simulink model "nav_closed_loop"  (R2026a)
settings: Solver=FixedStepDiscrete  StartTime=0  StopTime=182.32  FixedStep=Ts
values from neighbouring files (symbols this model uses):
  P = nav_params(cfg, root)    [build_nav_simulink.m]    (also in nav_ablation.m; nav_figures.m = PP; nav_main.m; nav_study.m)
  trk = struct('N', TR.trk.N, 'ds', TR.trk.ds, 'L', TR.trk.L, 'x', TR.trk.x, 'y', TR.trk.y,               'psi', TR.trk.psi, 'kap', TR.trk.kap)    [build_nav_simulink.m]    (also in nav_ablation.m = TR.trk; nav_figures.m = TR.trk; end; nav_main.m = TR.trk; track.mat = )
  Ts = P.T    [build_nav_simulink.m]
  xp0 = nav_plant_init(TR.trk, cfg.offset0)    [build_nav_simulink.m]
settings Model: ExtModeTrigDuration=10000  Creator=danielappel  LastModifiedBy=danielappel

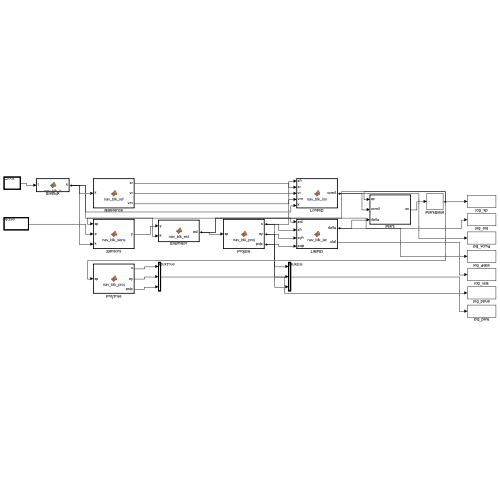
[thumbnail: Simulink's stored preview of the top-level diagram]
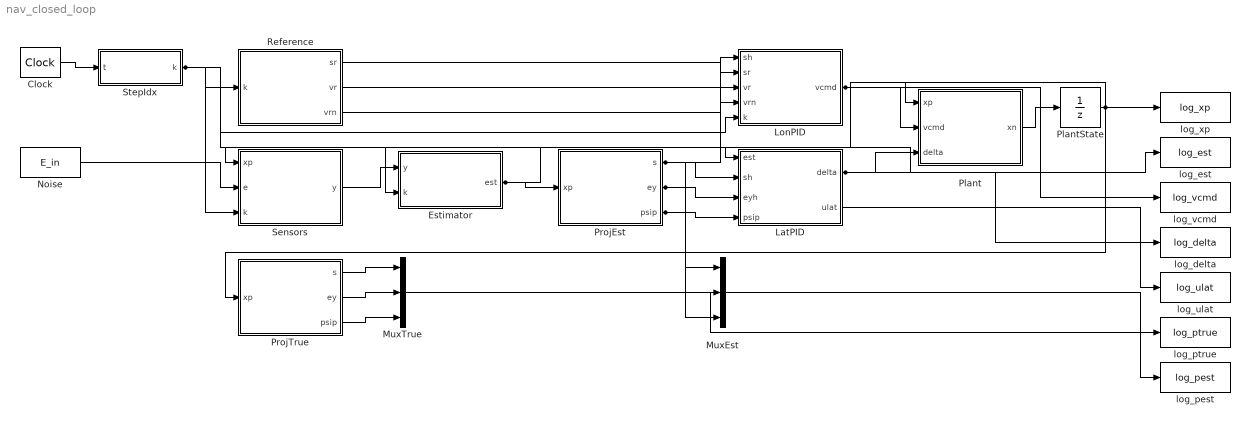
== system nav_closed_loop ==
  Clock : DigitalClock  SampleTime=Ts
  Estimator : MATLAB Function  TreatAsAtomicUnit=on
  LatPID : MATLAB Function  TreatAsAtomicUnit=on
  LonPID : MATLAB Function  TreatAsAtomicUnit=on
  MuxEst : Mux  Inputs=3
  MuxTrue : Mux  Inputs=3
  Noise : FromWorkspace  VariableName=E_in  SampleTime=Ts  Interpolate=off  OutputAfterFinalValue=Holding final value
  Plant : MATLAB Function  TreatAsAtomicUnit=on
  PlantState : UnitDelay  InitialCondition=xp0  SampleTime=Ts
  ProjEst : MATLAB Function  TreatAsAtomicUnit=on
  ProjTrue : MATLAB Function  TreatAsAtomicUnit=on
  Reference : MATLAB Function  TreatAsAtomicUnit=on
  Sensors : MATLAB Function  TreatAsAtomicUnit=on
  StepIdx : MATLAB Function  TreatAsAtomicUnit=on
  log_delta : ToWorkspace  VariableName=log_delta  SampleTime=Ts
  log_est : ToWorkspace  VariableName=log_est  SampleTime=Ts
  log_pest : ToWorkspace  VariableName=log_pest  SampleTime=Ts
  log_ptrue : ToWorkspace  VariableName=log_ptrue  SampleTime=Ts
  log_ulat : ToWorkspace  VariableName=log_ulat  SampleTime=Ts
  log_vcmd : ToWorkspace  VariableName=log_vcmd  SampleTime=Ts
  log_xp : ToWorkspace  VariableName=log_xp  SampleTime=Ts
  wires:
  Clock/1 -> StepIdx/1(t)
  StepIdx/1(k) -> Reference/1(k), Sensors/3(k), Estimator/2(k), LonPID/5(k)
  PlantState/1 -> Sensors/1(xp), ProjTrue/1(xp), Plant/1(xp), log_xp/1
  Noise/1 -> Sensors/2(e)
  Sensors/1(y) -> Estimator/1(y)
  Estimator/1(est) -> ProjEst/1(xp), LatPID/1(est), log_est/1
  ProjEst/1(s) -> LonPID/1(sh), LatPID/2(sh), MuxEst/1
  ProjEst/2(ey) -> LatPID/3(eyh), MuxEst/2
  ProjEst/3(psip) -> LatPID/4(psip), MuxEst/3
  Reference/1(sr) -> LonPID/2(sr)
  Reference/2(vr) -> LonPID/3(vr)
  Reference/3(vrn) -> LonPID/4(vrn)
  LonPID/1(vcmd) -> Plant/2(vcmd), log_vcmd/1
  LatPID/1(delta) -> Plant/3(delta), log_delta/1
  Plant/1(xn) -> PlantState/1
  LatPID/2(ulat) -> log_ulat/1
  ProjTrue/1(s) -> MuxTrue/1
  ProjTrue/2(ey) -> MuxTrue/2
  ProjTrue/3(psip) -> MuxTrue/3
  MuxTrue/1 -> log_ptrue/1
  MuxEst/1 -> log_pest/1

== matlab function nav_closed_loop/Reference ==
  data: k input; sr output double size=1; vr output double size=1; vrn output double size=1; REFF parameter
function [sr, vr, vrn] = nav_blk_ref(k, REFF)
n = numel(REFF.s);
i = min(max(round(k),1), n);
sr = REFF.s(i); vr = REFF.v(i); vrn = REFF.v(min(i+1,n));

== matlab function nav_closed_loop/StepIdx ==
  data: t input; k output double size=1; P parameter
function k = nav_blk_k(t, P)
k = round(t/P.T) + 1;

== matlab function nav_closed_loop/Sensors ==
  data: xp input; y output double size=8; e input; k input; P parameter
function y = nav_blk_sens(xp, e, k, P)
persistent vprev
if isempty(vprev), vprev = 0; end
[y, vprev] = nav_sensor_step(xp(:), vprev, e(:)', k, P);

== matlab function nav_closed_loop/Estimator ==
  data: y input; est output double size=7; k input; P parameter
function est = nav_blk_est(y, k, P)
persistent xs
if isempty(xs)
    xs = nav_est_init(P, P.xp0(1:2), P.xp0(3));
end
[xs, est] = nav_est_step(xs, y(:), k, P);

== matlab function nav_closed_loop/ProjEst ==
  data: xp input; s output double size=1; ey output double size=1; psip output double size=1; P parameter; trk parameter
function [s, ey, psip] = nav_blk_proj(xp, P, trk)
persistent ic
if isempty(ic), ic = 1; end
[s, ey, psip, ~, ic] = nav_project(xp(1), xp(2), ic, trk, P.W);

== matlab function nav_closed_loop/LonPID ==
  data: sh input; vcmd output double size=1; sr input; vr input; vrn input; k input; P parameter
function vcmd = nav_blk_lon(sh, sr, vr, vrn, k, P)
persistent ls
if isempty(ls), ls = nav_lon_init(); end
[vcmd, ls] = nav_lon_step(ls, sh, sr, vr, vrn, double(k > P.nst), P);

== matlab function nav_closed_loop/LatPID ==
  data: est input; delta output double size=1; sh input; eyh input; psip input; ulat output double size=1; P parameter; trk parameter
function [delta, ulat] = nav_blk_lat(est, sh, eyh, psip, P, trk)
persistent ls
if isempty(ls), ls = nav_lat_init(); end
vh = hypot(est(3), est(4));
[delta, ls, ulat] = nav_lat_step(ls, eyh, vh, sh, psip, est(3:4), trk, P);

== matlab function nav_closed_loop/Plant ==
  data: xp input; xn output double size=9; vcmd input; delta input; P parameter
function xn = nav_blk_plant(xp, vcmd, delta, P)
xn = nav_plant_step(xp(:), vcmd, delta, P);

== matlab function nav_closed_loop/ProjTrue ==
  data: xp input; s output double size=1; ey output double size=1; psip output double size=1; P parameter; trk parameter
function [s, ey, psip] = nav_blk_proj(xp, P, trk)
persistent ic
if isempty(ic), ic = 1; end
[s, ey, psip, ~, ic] = nav_project(xp(1), xp(2), ic, trk, P.W);
